simulink model "rov_ctrl_deploy"  (R2023b)
settings: Solver=FixedStepDiscrete  StartTime=0  StopTime=100  FixedStep=0.01  RelTol=1e-3
PreLoadFcn:
  | try, S=load('rovmodel75kg.mat'); catch, S=load('C:\Users\yhm\wb_hil\rovmodel75kg.mat'); end; fn=fieldnames(S); for k=1:numel(fn), assignin('base',fn{k},S.(fn{k})); end; M_nom=S.M; Ma_nom=S.Ma; DL_nom=S.DL; clear S fn k;
values from neighbouring files (symbols this model uses):
  I = [2.51  0  0; 0  3.38  0.01; 0  0.01  1.73]    [rovmodel75kg.mat]
  m = [75  0  0; 0  75  0; 0  0  75]    [rovmodel75kg.mat]
  Ma = [-20.392 0 0 0 0 0 0 -53.435 0 0 0 0 ... (36 elements, 6x6)]    [rovmodel75kg.mat]
  rg = [0 0 0]    [rovmodel75kg.mat]
undefined symbols (not defined in the file or in its folder): DiscIntNeverNeededParam
libraries: matrix_library x6, simulink x1
settings Model: Creator=yhm  LastModifiedBy=yhm
settings OptimizationCC: DefaultParameterBehavior=Inlined  EnhancedBackFolding=on  PassReuseOutputArgsAs=Individual arguments  ZeroExternalMemoryAtStartup=off  ZeroInternalMemoryAtStartup=off  OptimizeBlockOrder=speed  DifferentSizesBufferReuse=on  OptimizationCustomize=off  EfficientTunableParamExpr=on
settings DebuggingCC: ParameterTunabilityLossMsg=error
settings SFSimCC: MATLABDynamicMemAlloc=off
settings RTWCC: Description=Embedded Coder  SystemTargetFile=ert.tlc  TemplateMakefile=ert_default_tmf
settings CodeAppCC: ForceParamTrailComments=on  IgnoreCustomStorageClasses=off  OperatorAnnotations=on  SimulinkDataObjDesc=on  SFDataObjDesc=on  InsertBlockDesc=on
settings ERTTargetCC: TargetLangStandard=C99 (ISO)  GenerateSampleERTMain=on  InlinedParameterPlacement=NonHierarchical  ERTCustomFileTemplate=example_file_process.tlc

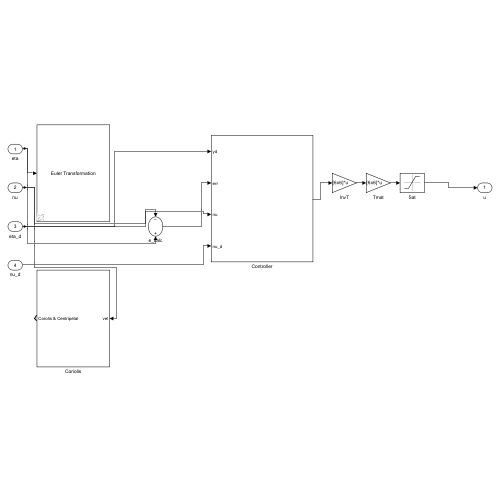
[thumbnail: Simulink's stored preview of the top-level diagram]
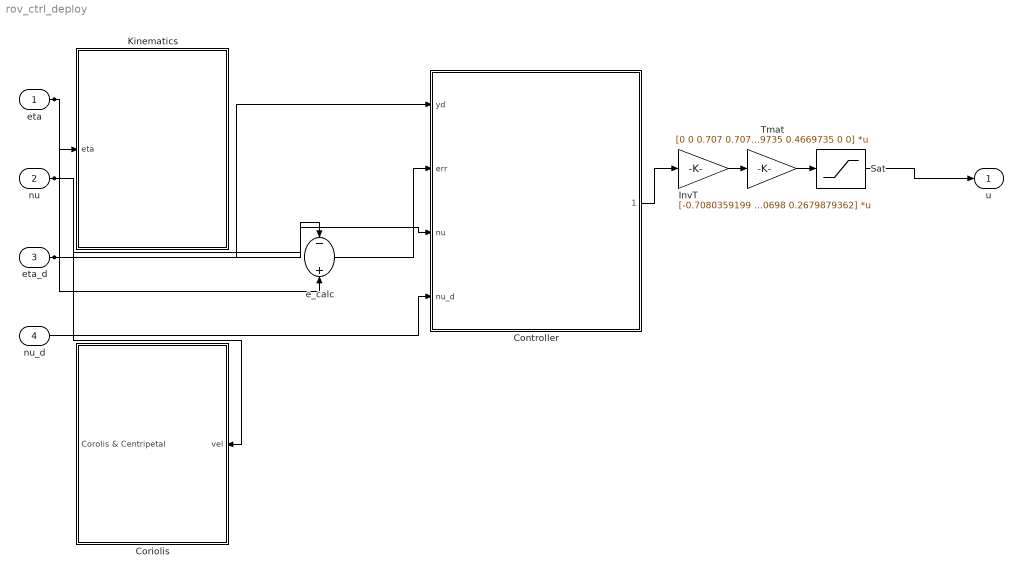
== system rov_ctrl_deploy ==
  eta : Inport  OutDataTypeStr=double  PortDimensions=6
  nu : Inport  Port=2  OutDataTypeStr=double  PortDimensions=6
  eta_d : Inport  Port=3  OutDataTypeStr=double  PortDimensions=6
  nu_d : Inport  Port=4  OutDataTypeStr=double  PortDimensions=6
  Controller : Subsystem
  Coriolis : Subsystem
  InvT : Gain  Gain=[-0.7080359199 -0.4427626243 0.05838623729 9.795787713e-17 1.644682741 -0.6703446242;-0.7080359199 0.4427626243 0.05838623729 3.755136333e-16 1.644682741 0.6703446242;0.7072135785 0.2644509542 1.700029006e-16 3.936371478e-16 -9.992007222e-16 -0.6703446242;0.7072135785 -0.2644509542 4.510281038e-17 1.299591795e-16 -1.054711873e-15 0.6703446242;0.5005813953 -0.1770060319 0.4587209302 -1.818181818 -1.162790698 -0.2679879362;0.5005813953 0.1770060319 0.4587209302 1.818181818 -1.162790698 0.2679879362]  Multiplication=Matrix(K*u)
  Kinematics : Subsystem  AncestorBlock=rov_design_analysis/Scope Utilities/Euler Transformation
      mask Display: disp('Euler Transformation')
  Sat : Saturate  UpperLimit=100  LowerLimit=-100
  Tmat : Gain  Gain=[0 0 0.707 0.707 0 0;-0.707 0.707 0.707 -0.707 0 0;0.707 0.707 0 0 1 1;0.1099385 -0.1099385 0 0 -0.275 0.275;0.2789115 0.2789115 0.3043635 0.3043635 -0.0355 -0.0355;-0.2789115 0.2789115 -0.4669735 0.4669735 0 0]  Multiplication=Matrix(K*u)
  e_calc : Sum  Inputs=-+
  u : Outport  PortDimensions=6
  wires:
  eta/1 -> Kinematics/1(eta), e_calc/2
  nu/1 -> Coriolis/1(vel), Controller/3(nu)
  eta_d/1 -> e_calc/1, Controller/1(yd)
  nu_d/1 -> Controller/4(nu_d)
  e_calc/1 -> Controller/2(err)
  Controller/1(" ") -> InvT/1
  InvT/1 -> Tmat/1
  Tmat/1 -> Sat/1
  Sat/1 -> u/1

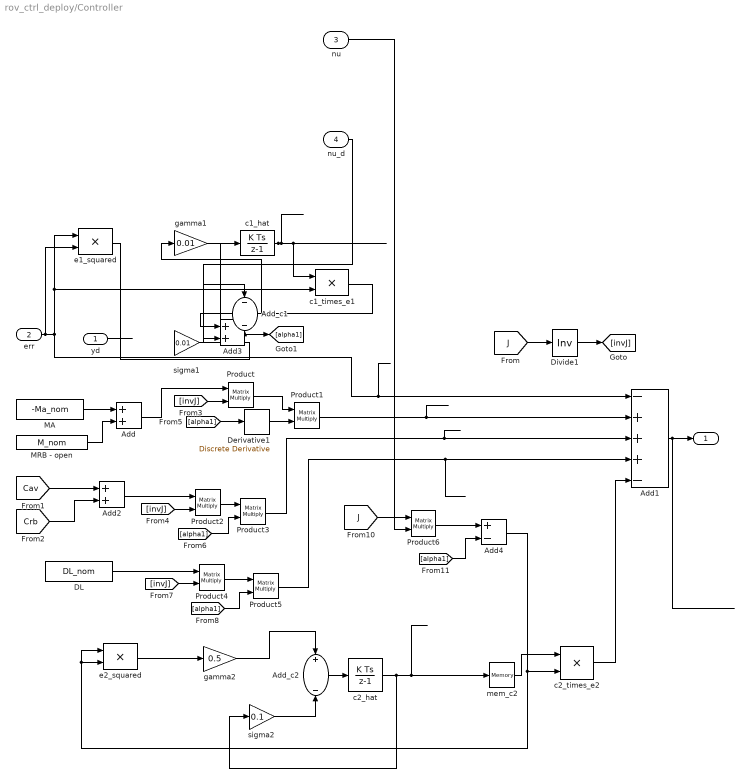
== system rov_ctrl_deploy/Controller ==
  yd : Inport  PortDimensions=6
  err : Inport  Port=2  PortDimensions=6
  nu : Inport  Port=3  OutDataTypeStr=double  PortDimensions=6
  nu_d : Inport  Port=4  OutDataTypeStr=double  PortDimensions=6
  Add : Sum
  Add1 : Sum  Inputs=-+++-
  Add2 : Sum
  Add3 : Sum
  Add4 : Sum  Inputs=+-
  Add_c1 : Sum  Inputs=--
  Add_c2 : Sum  Inputs=+-
  DL : Constant  Value=DL_nom
  Derivative1 : simulink/Discrete/Discrete Derivative  gainval=1  ICPrevScaledInput=0.0  OutMin=[]  OutMax=[]  OutDataType=fixdt(1, 16)  OutScaling=2^-10  DoSatur=off
      link override UD: SampleTime=0.01
  Divide1 : Product  Inputs=/  Multiplication=Matrix(*)
  MA : Constant  Value=-Ma_nom
  MRB - open : Constant  Value=M_nom
  Product{,1..6} (7 alike) : Product  Multiplication=Matrix(*)
  c1_hat : DiscreteIntegrator  InitialCondition=-3  SampleTime=0.01  ICPrevOutput=DiscIntNeverNeededParam  ICPrevScaledInput=DiscIntNeverNeededParam
  c1_times_e1 : Product
  c2_hat : DiscreteIntegrator  InitialCondition=5  SampleTime=0.01  ICPrevOutput=DiscIntNeverNeededParam  ICPrevScaledInput=DiscIntNeverNeededParam
  c2_times_e2 : Product
  e1_squared : Product
  e2_squared : Product
  gamma1 : Gain  Gain=0.01
  gamma2 : Gain  Gain=0.5
  mem_c2 : Memory  InitialCondition=5
  sigma1 : Gain  Gain=0.01
  sigma2 : Gain  Gain=0.1
  " " : Outport  PortDimensions=6
  wires:
  gamma1/1 -> c1_hat/1
  Add_c1/1 -> gamma1/1
  e1_squared/1 -> Add_c1/2
  sigma1/1 -> Add_c1/1
  c2_hat/1 -> sigma2/1, mem_c2/1
  e2_squared/1 -> gamma2/1
  mem_c2/1 -> c2_times_e2/1
  Add4/1 -> c2_times_e2/2, e2_squared/2, e2_squared/1
  c2_times_e2/1 -> Add1/5
  Add1/1 -> " "/1
  c1_times_e1/1 -> Add3/1
  Add_c2/1 -> c2_hat/1
  sigma2/1 -> Add_c2/2
  gamma2/1 -> Add_c2/1
  c1_hat/1 -> sigma1/1, c1_times_e1/1
  err/1 -> e1_squared/2, Add1/1, c1_times_e1/2, e1_squared/1
  Product1/1 -> Add1/2
  Product3/1 -> Add1/3
  Product5/1 -> Add1/4
  [alpha1] -> Add4/2
  Product6/1 -> Add4/1
  [J] -> Product6/1
  [alpha1] -> Product5/2
  Product4/1 -> Product5/1
  [invJ] -> Product4/2
  DL/1 -> Product4/1
  [alpha1] -> Derivative1/1
  Derivative1/1 -> Product1/2
  [alpha1] -> Product3/2
  Add3/1 -> [alpha1]
  Product2/1 -> Product3/1
  [invJ] -> Product2/2
  Add2/1 -> Product2/1
  [invJ] -> Product/2
  Divide1/1 -> [invJ]
  [Cav] -> Add2/1
  [Crb] -> Add2/2
  Product/1 -> Product1/1
  yd/1 -> ?
  Add/1 -> Product/1
  [J] -> Divide1/1
  MRB - open/1 -> Add/2
  MA/1 -> Add/1
  nu/1 -> Product6/2
  nu_d/1 -> Add3/2

== system rov_ctrl_deploy/Coriolis ==
  vel : Inport
  Add2 : Sum
  Centripetal & Coriolis : Subsystem  AncestorBlock=rov_design_analysis/ROV Models/1. Six DOF RRC ROV II/Centripetal & Coriolis
      mask Display: disp('CRB')
  Centripetal & Coriolis1 : Subsystem  AncestorBlock=rov_design_analysis/ROV Models/1. Six DOF RRC ROV II/Centripetal & Coriolis
      mask Display: disp('CA')
  Product5 : Product  Multiplication=Matrix(*)
  Subsystem : Subsystem
      mask Display: disp('CRB(v)')
  Corolis & Centripetal : Outport
  tag scope: Cav=global, Crb=global
  wires:
  Centripetal & Coriolis1/1(Ca) -> Add2/1, [Cav]
  Subsystem/1(Out1) -> [Crb], Add2/2
  Product5/1 -> Corolis & Centripetal/1
  vel/1 -> Centripetal & Coriolis1/1(vel), Subsystem/1(In1), Product5/2
  Add2/1 -> Product5/1

== system rov_ctrl_deploy/Kinematics ==
  eta : Inport
  Demux1 : Demux  Outputs=2
      settings: DisplayOption=none
  Matrix Concatenate6 : Concatenate  NumInputs=6  Mode=Multidimensional array
  Subsystem : Subsystem
      mask Display: disp('Transformation J first Row')
  Subsystem1 : Subsystem
      mask Display: disp('Transformation J second Row')
  Subsystem2 : Subsystem
      mask Display: disp('Transformation J third Row')
  Subsystem3 : Subsystem
      mask Display: disp('Transformation J fourth Row')
  Subsystem4 : Subsystem
      mask Display: disp('Transformation J fifth Row')
  Subsystem5 : Subsystem
      mask Display: disp('Transformation J sixth Row')
  tag scope: J=global
  wires:
  ? -> ?
  ? -> ?
  Subsystem5/1(Out1) -> Matrix Concatenate6/6
  Subsystem4/1(Out1) -> Matrix Concatenate6/5
  Subsystem3/1(Out1) -> Matrix Concatenate6/4
  Subsystem2/1(Out1) -> Matrix Concatenate6/3
  Subsystem1/1(Out1) -> Matrix Concatenate6/2
  Demux1/2 -> Subsystem5/1(In1), Subsystem4/1(In1), Subsystem3/1(In1), Subsystem2/1(In1), Subsystem1/1(In1), Subsystem/1(In1)
  Subsystem/1(Out1) -> Matrix Concatenate6/1
  Matrix Concatenate6/1 -> [J]
  ? -> ?
  Demux1/1 -> ?
  eta/1 -> Demux1/1

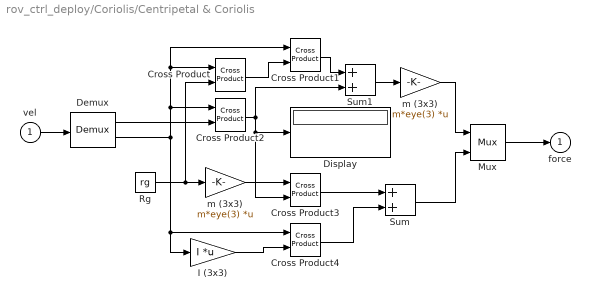
== system rov_ctrl_deploy/Coriolis/Centripetal & Coriolis ==
  vel : Inport
  Cross Product{,1..4} (5 alike) : matrix_library/Cross Product
  Demux : Demux  Outputs=2
      settings: DisplayOption=none
  Display : Display
  "I (3x3) " : Gain  Gain=I  Multiplication=Matrix(K*u)  SaturateOnIntegerOverflow=on  OutDataTypeStr=Inherit: Same as input  ParamDataTypeStr=Inherit: Same as input
  Mux : Mux  Inputs=2
  Rg : Constant  Value=rg
  Sum : Sum  InputSameDT=on  SaturateOnIntegerOverflow=on  OutDataTypeStr=Inherit: Same as first input
  Sum1 : Sum  InputSameDT=on  SaturateOnIntegerOverflow=on  OutDataTypeStr=Inherit: Same as first input
  m (3x3) : Gain  Gain=m*eye(3)  Multiplication=Matrix(K*u)  SaturateOnIntegerOverflow=on  OutDataTypeStr=Inherit: Same as input  ParamDataTypeStr=Inherit: Same as input
  "m (3x3) " : Gain  Gain=m*eye(3)  Multiplication=Matrix(K*u)  SaturateOnIntegerOverflow=on  OutDataTypeStr=Inherit: Same as input  ParamDataTypeStr=Inherit: Same as input
  force : Outport  InitialOutput=0
  wires:
  Demux/1 -> Cross Product2/2
  Cross Product2/1 -> Sum1/2, Display/1, Cross Product3/2
  "I (3x3) "/1 -> Cross Product4/2
  Rg/1 -> "m (3x3) "/1, Cross Product/2
  Demux/2 -> "I (3x3) "/1, Cross Product4/1, Cross Product/1, Cross Product1/1, Cross Product2/1
  Mux/1 -> force/1
  Sum/1 -> Mux/2
  m (3x3)/1 -> Mux/1
  vel/1 -> Demux/1
  Sum1/1 -> m (3x3)/1
  Cross Product1/1 -> Sum1/1
  Cross Product/1 -> Cross Product1/2
  Cross Product3/1 -> Sum/1
  "m (3x3) "/1 -> Cross Product3/1
  Cross Product4/1 -> Sum/2

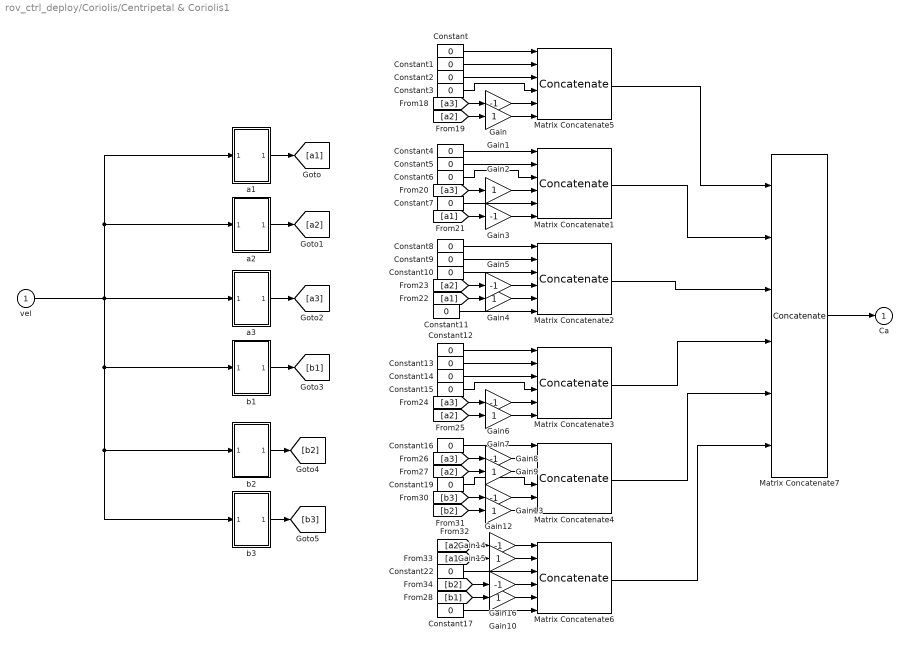
== system rov_ctrl_deploy/Coriolis/Centripetal & Coriolis1 ==
  vel : Inport
  Constant{,1..17,19,22} (20 alike) : Constant  Value=0
  Gain{,3,5..6,8,12,14,16} (8 alike) : Gain  Gain=-1
  Gain{1..2,4,7,9..10,13,15} (8 alike) : Gain
  Matrix Concatenate{1..6} (6 alike) : Concatenate  NumInputs=6  Mode=Multidimensional array  ConcatenateDimension=2
  Matrix Concatenate7 : Concatenate  NumInputs=6  Mode=Multidimensional array
  a1 : Subsystem
      mask Display: disp('Row 1')
  a2 : Subsystem
      mask Display: disp('Row 2')
  a3 : Subsystem
      mask Display: disp('Row 1')
  b1 : Subsystem
      mask Display: disp('Row 2')
  b2 : Subsystem
      mask Display: disp('Row 1')
  b3 : Subsystem
      mask Display: disp('Row 2')
  Ca : Outport  InitialOutput=0
  wires:
  Matrix Concatenate7/1 -> Ca/1
  Matrix Concatenate6/1 -> Matrix Concatenate7/6
  Matrix Concatenate4/1 -> Matrix Concatenate7/5
  Matrix Concatenate3/1 -> Matrix Concatenate7/4
  Matrix Concatenate2/1 -> Matrix Concatenate7/3
  Matrix Concatenate1/1 -> Matrix Concatenate7/2
  Matrix Concatenate5/1 -> Matrix Concatenate7/1
  Constant17/1 -> Matrix Concatenate6/6
  [b2] -> Gain16/1
  Gain16/1 -> Matrix Concatenate6/4
  [a1] -> Gain15/1
  Gain15/1 -> Matrix Concatenate6/2
  [a2] -> Gain14/1
  Gain14/1 -> Matrix Concatenate6/1
  [b2] -> Gain13/1
  Gain13/1 -> Matrix Concatenate4/6
  Gain12/1 -> Matrix Concatenate4/5
  [b3] -> Gain12/1
  Gain9/1 -> Matrix Concatenate4/3
  Constant11/1 -> Matrix Concatenate2/6
  Gain5/1 -> Matrix Concatenate2/4
  Constant7/1 -> Matrix Concatenate1/5
  Constant6/1 -> Matrix Concatenate1/3
  Gain2/1 -> Matrix Concatenate1/4
  Gain10/1 -> Matrix Concatenate6/5
  [b1] -> Gain10/1
  Constant22/1 -> Matrix Concatenate6/3
  Constant16/1 -> Matrix Concatenate4/1
  [a2] -> Gain9/1
  Constant19/1 -> Matrix Concatenate4/4
  [a3] -> Gain8/1
  Gain8/1 -> Matrix Concatenate4/2
  Constant12/1 -> Matrix Concatenate3/1
  Gain6/1 -> Matrix Concatenate3/5
  Gain7/1 -> Matrix Concatenate3/6
  [a2] -> Gain7/1
  Constant15/1 -> Matrix Concatenate3/4
  [a3] -> Gain6/1
  Constant13/1 -> Matrix Concatenate3/2
  Constant14/1 -> Matrix Concatenate3/3
  Constant8/1 -> Matrix Concatenate2/1
  Gain4/1 -> Matrix Concatenate2/5
  [a2] -> Gain5/1
  [a1] -> Gain4/1
  Constant9/1 -> Matrix Concatenate2/2
  Constant10/1 -> Matrix Concatenate2/3
  Constant4/1 -> Matrix Concatenate1/1
  Gain3/1 -> Matrix Concatenate1/6
  [a1] -> Gain3/1
  [a3] -> Gain2/1
  Constant5/1 -> Matrix Concatenate1/2
  [a2] -> Gain1/1
  [a3] -> Gain/1
  Constant3/1 -> Matrix Concatenate5/4
  Constant2/1 -> Matrix Concatenate5/3
  Constant1/1 -> Matrix Concatenate5/2
  Gain1/1 -> Matrix Concatenate5/6
  Gain/1 -> Matrix Concatenate5/5
  Constant/1 -> Matrix Concatenate5/1
  b3/1(Out1) -> [b3]
  b1/1(Out1) -> [b1]
  a2/1(Out1) -> [a2]
  a3/1(Out1) -> [a3]
  b2/1(Out1) -> [b2]
  a1/1(Out1) -> [a1]
  vel/1 -> a2/1(In1), a1/1(In1), a3/1(In1), b1/1(In1), b2/1(In1), b3/1(In1)

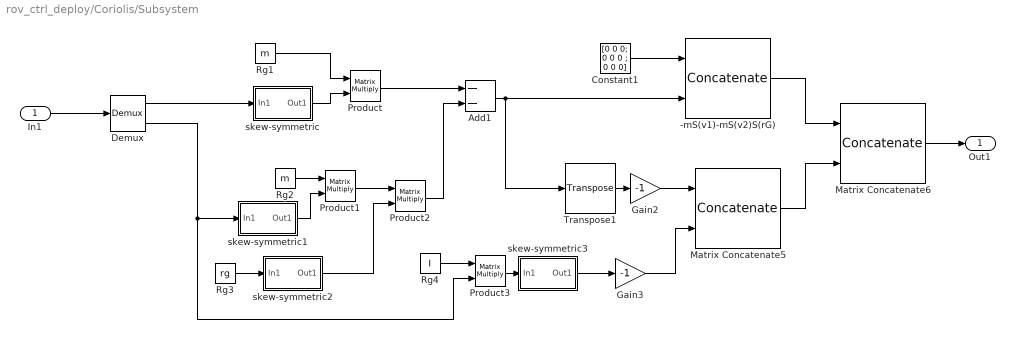
== system rov_ctrl_deploy/Coriolis/Subsystem ==
  In1 : Inport
  -mS(v1)-mS(v2)S(rG) : Concatenate  Mode=Multidimensional array  ConcatenateDimension=2
  Add1 : Sum  Inputs=--
  Constant1 : Constant  Value=[0 0 0; 0 0 0 ; 0 0 0]
  Demux : Demux  Outputs=2
      settings: DisplayOption=none
  Gain2 : Gain  Gain=-1
  Gain3 : Gain  Gain=-1
  Matrix Concatenate5 : Concatenate  Mode=Multidimensional array  ConcatenateDimension=2
  Matrix Concatenate6 : Concatenate  Mode=Multidimensional array
  Product{,1..3} (4 alike) : Product  Multiplication=Matrix(*)
  Rg1 : Constant  Value=m
  Rg2 : Constant  Value=m
  Rg3 : Constant  Value=rg
  Rg4 : Constant  Value=I
  Transpose1 : matrix_library/Transpose
  skew-symmetric : Subsystem
  skew-symmetric1 : Subsystem
  skew-symmetric2 : Subsystem
  skew-symmetric3 : Subsystem
  Out1 : Outport
  wires:
  Product1/1 -> Product2/1
  Product/1 -> Add1/1
  Rg1/1 -> Product/1
  -mS(v1)-mS(v2)S(rG)/1 -> Matrix Concatenate6/1
  Demux/1 -> skew-symmetric/1(In1)
  skew-symmetric/1(Out1) -> Product/2
  skew-symmetric2/1(Out1) -> Product2/2
  Transpose1/1 -> Gain2/1
  skew-symmetric3/1(Out1) -> Gain3/1
  Matrix Concatenate6/1 -> Out1/1
  Gain2/1 -> Matrix Concatenate5/1
  Product2/1 -> Add1/2
  Add1/1 -> Transpose1/1, -mS(v1)-mS(v2)S(rG)/2
  Gain3/1 -> Matrix Concatenate5/2
  Demux/2 -> skew-symmetric1/1(In1), Product3/2
  Constant1/1 -> -mS(v1)-mS(v2)S(rG)/1
  Rg4/1 -> Product3/1
  Matrix Concatenate5/1 -> Matrix Concatenate6/2
  Rg3/1 -> skew-symmetric2/1(In1)
  skew-symmetric1/1(Out1) -> Product1/2
  Product3/1 -> skew-symmetric3/1(In1)
  Rg2/1 -> Product1/1
  In1/1 -> Demux/1

== system rov_ctrl_deploy/Kinematics/Subsystem ==
  In1 : Inport
  -sZ.cX+cZ.sY.sX : Fcn  Expr=-sin(u[3])*cos(u[1]) + cos(u[3])*sin(u[2])*sin(u[1])
  Constant : Constant  Value=0
  Matrix Concatenate : Concatenate  NumInputs=6  Mode=Multidimensional array  ConcatenateDimension=2
  cY.cZ : Fcn  Expr=cos(u[3]) * cos(u[2])
  sZ.sX+cZ.cX.sY : Fcn  Expr=sin(u[3])*sin(u[1]) + cos(u[3])*cos(u[1])*sin(u[2])
  Out1 : Outport
  wires:
  In1/1 -> cY.cZ/1, -sZ.cX+cZ.sY.sX/1, sZ.sX+cZ.cX.sY/1
  -sZ.cX+cZ.sY.sX/1 -> Matrix Concatenate/2
  sZ.sX+cZ.cX.sY/1 -> Matrix Concatenate/3
  Matrix Concatenate/1 -> Out1/1
  cY.cZ/1 -> Matrix Concatenate/1
  Constant/1 -> Matrix Concatenate/4, Matrix Concatenate/5, Matrix Concatenate/6

== system rov_ctrl_deploy/Kinematics/Subsystem1 ==
  In1 : Inport
  -cZ.sX+sY.sZ.cX : Fcn  Expr=-cos(u[3])*sin(u[1]) + sin(u[2])*sin(u[3])*cos(u[1])
  Constant1 : Constant  Value=0
  Matrix Concatenate1 : Concatenate  NumInputs=6  Mode=Multidimensional array  ConcatenateDimension=2
  cY.sZ : Fcn  Expr=sin(u[3]) * cos(u[2])
  cZ.cX+sX.sY.sZ : Fcn  Expr=cos(u[3])*cos(u[1]) + sin(u[1])*sin(u[2])*sin(u[3])
  Out1 : Outport
  wires:
  In1/1 -> cY.sZ/1, cZ.cX+sX.sY.sZ/1, -cZ.sX+sY.sZ.cX/1
  Constant1/1 -> Matrix Concatenate1/4, Matrix Concatenate1/5, Matrix Concatenate1/6
  cZ.cX+sX.sY.sZ/1 -> Matrix Concatenate1/2
  -cZ.sX+sY.sZ.cX/1 -> Matrix Concatenate1/3
  Matrix Concatenate1/1 -> Out1/1
  cY.sZ/1 -> Matrix Concatenate1/1

== system rov_ctrl_deploy/Kinematics/Subsystem2 ==
  In1 : Inport
  -sY : Fcn  Expr=-sin(u[2])
  Constant2 : Constant  Value=0
  Matrix Concatenate2 : Concatenate  NumInputs=6  Mode=Multidimensional array  ConcatenateDimension=2
  cY.cX : Fcn  Expr=cos(u[2])*cos(u[1])
  cY.sX : Fcn  Expr=cos(u[2])*sin(u[1])
  Out1 : Outport
  wires:
  In1/1 -> -sY/1, cY.sX/1, cY.cX/1
  -sY/1 -> Matrix Concatenate2/1
  cY.cX/1 -> Matrix Concatenate2/3
  cY.sX/1 -> Matrix Concatenate2/2
  Constant2/1 -> Matrix Concatenate2/4, Matrix Concatenate2/5, Matrix Concatenate2/6
  Matrix Concatenate2/1 -> Out1/1

== system rov_ctrl_deploy/Kinematics/Subsystem3 ==
  In1 : Inport
  1 : Fcn  Expr=1
  Constant3 : Constant  Value=0
  Matrix Concatenate3 : Concatenate  NumInputs=6  Mode=Multidimensional array  ConcatenateDimension=2
  cX.tY : Fcn  Expr=cos(u[1])*tan(u[2])
  sX.tY : Fcn  Expr=sin(u[1])*tan(u[2])
  Out1 : Outport
  wires:
  In1/1 -> 1/1, sX.tY/1, cX.tY/1
  Matrix Concatenate3/1 -> Out1/1
  Constant3/1 -> Matrix Concatenate3/1, Matrix Concatenate3/2, Matrix Concatenate3/3
  1/1 -> Matrix Concatenate3/4
  sX.tY/1 -> Matrix Concatenate3/5
  cX.tY/1 -> Matrix Concatenate3/6

== system rov_ctrl_deploy/Kinematics/Subsystem4 ==
  In1 : Inport
  -sX : Fcn  Expr=-sin(u[1])
  0 : Fcn  Expr=0
  Constant4 : Constant  Value=0
  Dot Product1 : Subsystem
  Matrix Concatenate4 : Concatenate  NumInputs=6  Mode=Multidimensional array  ConcatenateDimension=2
  cX : Fcn  Expr=cos(u[1])
  Out1 : Outport
  wires:
  -sX/1 -> Matrix Concatenate4/6
  Constant4/1 -> Matrix Concatenate4/1, Matrix Concatenate4/2, Matrix Concatenate4/3
  Matrix Concatenate4/1 -> Out1/1
  0/1 -> Matrix Concatenate4/4
  cX/1 -> Matrix Concatenate4/5
  In1/1 -> 0/1, cX/1, -sX/1

== system rov_ctrl_deploy/Kinematics/Subsystem5 ==
  In1 : Inport
  2 : Fcn  Expr=0
  Constant5 : Constant  Value=0
  Matrix Concatenate5 : Concatenate  NumInputs=6  Mode=Multidimensional array  ConcatenateDimension=2
  cX/cY : Fcn  Expr=cos(u[1])/cos(u[2])
  sX/cY : Fcn  Expr=sin(u[1])/cos(u[2])
  Out1 : Outport
  wires:
  Matrix Concatenate5/1 -> Out1/1
  sX/cY/1 -> Matrix Concatenate5/5
  2/1 -> Matrix Concatenate5/4
  In1/1 -> 2/1, sX/cY/1, cX/cY/1
  cX/cY/1 -> Matrix Concatenate5/6
  Constant5/1 -> Matrix Concatenate5/1, Matrix Concatenate5/2, Matrix Concatenate5/3

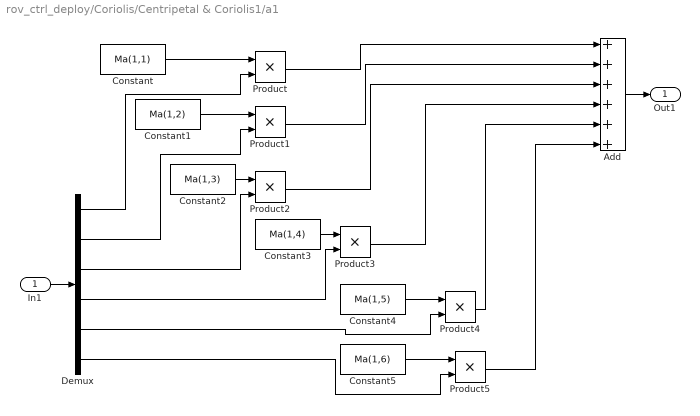
== system rov_ctrl_deploy/Coriolis/Centripetal & Coriolis1/a1 ==
  In1 : Inport
  Add : Sum  Inputs=++++++
  Constant : Constant  Value=Ma(1,1)
  Constant1 : Constant  Value=Ma(1,2)
  Constant2 : Constant  Value=Ma(1,3)
  Constant3 : Constant  Value=Ma(1,4)
  Constant4 : Constant  Value=Ma(1,5)
  Constant5 : Constant  Value=Ma(1,6)
  Demux : Demux  Outputs=6
  Product{,1..5} (6 alike) : Product  RndMeth=Zero
  Out1 : Outport
  wires:
  In1/1 -> Demux/1
  Add/1 -> Out1/1
  Constant/1 -> Product/1
  Product/1 -> Add/1
  Constant1/1 -> Product1/1
  Product1/1 -> Add/2
  Constant2/1 -> Product2/1
  Product2/1 -> Add/3
  Constant3/1 -> Product3/1
  Product3/1 -> Add/4
  Constant4/1 -> Product4/1
  Product4/1 -> Add/5
  Constant5/1 -> Product5/1
  Product5/1 -> Add/6
  Demux/6 -> Product5/2
  Demux/5 -> Product4/2
  Demux/4 -> Product3/2
  Demux/3 -> Product2/2
  Demux/2 -> Product1/2
  Demux/1 -> Product/2

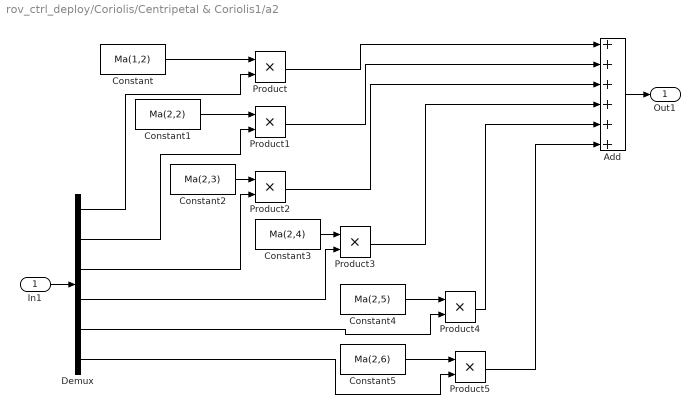
== system rov_ctrl_deploy/Coriolis/Centripetal & Coriolis1/a2 ==
  In1 : Inport
  Add : Sum  Inputs=++++++
  Constant : Constant  Value=Ma(1,2)
  Constant1 : Constant  Value=Ma(2,2)
  Constant2 : Constant  Value=Ma(2,3)
  Constant3 : Constant  Value=Ma(2,4)
  Constant4 : Constant  Value=Ma(2,5)
  Constant5 : Constant  Value=Ma(2,6)
  Demux : Demux  Outputs=6
  Product{,1..5} (6 alike) : Product  RndMeth=Zero
  Out1 : Outport
  wires:
  In1/1 -> Demux/1
  Add/1 -> Out1/1
  Constant/1 -> Product/1
  Product/1 -> Add/1
  Constant1/1 -> Product1/1
  Product1/1 -> Add/2
  Constant2/1 -> Product2/1
  Product2/1 -> Add/3
  Constant3/1 -> Product3/1
  Product3/1 -> Add/4
  Constant4/1 -> Product4/1
  Product4/1 -> Add/5
  Constant5/1 -> Product5/1
  Product5/1 -> Add/6
  Demux/6 -> Product5/2
  Demux/5 -> Product4/2
  Demux/4 -> Product3/2
  Demux/3 -> Product2/2
  Demux/2 -> Product1/2
  Demux/1 -> Product/2

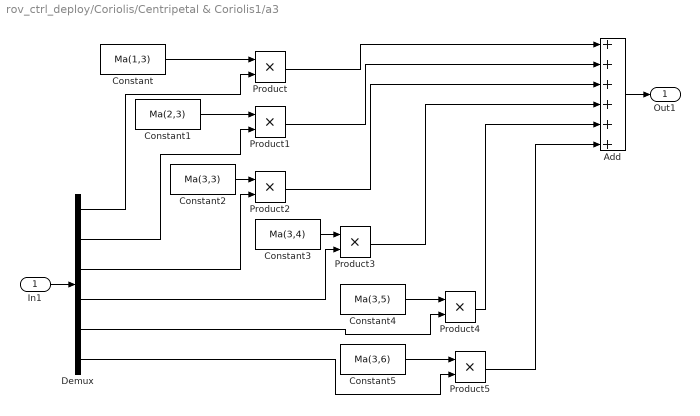
== system rov_ctrl_deploy/Coriolis/Centripetal & Coriolis1/a3 ==
  In1 : Inport
  Add : Sum  Inputs=++++++
  Constant : Constant  Value=Ma(1,3)
  Constant1 : Constant  Value=Ma(2,3)
  Constant2 : Constant  Value=Ma(3,3)
  Constant3 : Constant  Value=Ma(3,4)
  Constant4 : Constant  Value=Ma(3,5)
  Constant5 : Constant  Value=Ma(3,6)
  Demux : Demux  Outputs=6
  Product{,1..5} (6 alike) : Product  RndMeth=Zero
  Out1 : Outport
  wires:
  In1/1 -> Demux/1
  Add/1 -> Out1/1
  Constant/1 -> Product/1
  Product/1 -> Add/1
  Constant1/1 -> Product1/1
  Product1/1 -> Add/2
  Constant2/1 -> Product2/1
  Product2/1 -> Add/3
  Constant3/1 -> Product3/1
  Product3/1 -> Add/4
  Constant4/1 -> Product4/1
  Product4/1 -> Add/5
  Constant5/1 -> Product5/1
  Product5/1 -> Add/6
  Demux/6 -> Product5/2
  Demux/5 -> Product4/2
  Demux/4 -> Product3/2
  Demux/3 -> Product2/2
  Demux/2 -> Product1/2
  Demux/1 -> Product/2

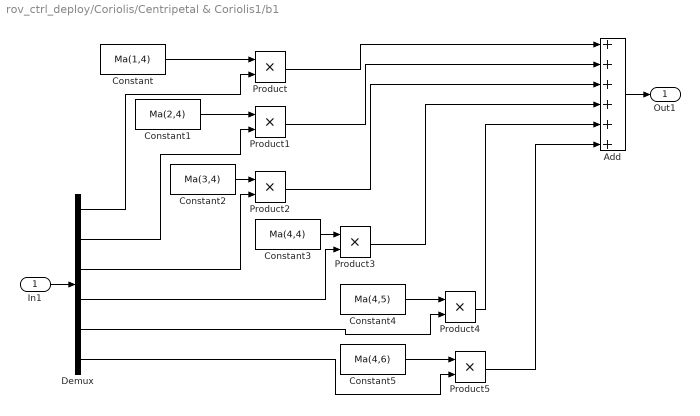
== system rov_ctrl_deploy/Coriolis/Centripetal & Coriolis1/b1 ==
  In1 : Inport
  Add : Sum  Inputs=++++++
  Constant : Constant  Value=Ma(1,4)
  Constant1 : Constant  Value=Ma(2,4)
  Constant2 : Constant  Value=Ma(3,4)
  Constant3 : Constant  Value=Ma(4,4)
  Constant4 : Constant  Value=Ma(4,5)
  Constant5 : Constant  Value=Ma(4,6)
  Demux : Demux  Outputs=6
  Product{,1..5} (6 alike) : Product  RndMeth=Zero
  Out1 : Outport
  wires:
  In1/1 -> Demux/1
  Add/1 -> Out1/1
  Constant/1 -> Product/1
  Product/1 -> Add/1
  Constant1/1 -> Product1/1
  Product1/1 -> Add/2
  Constant2/1 -> Product2/1
  Product2/1 -> Add/3
  Constant3/1 -> Product3/1
  Product3/1 -> Add/4
  Constant4/1 -> Product4/1
  Product4/1 -> Add/5
  Constant5/1 -> Product5/1
  Product5/1 -> Add/6
  Demux/6 -> Product5/2
  Demux/5 -> Product4/2
  Demux/4 -> Product3/2
  Demux/3 -> Product2/2
  Demux/2 -> Product1/2
  Demux/1 -> Product/2

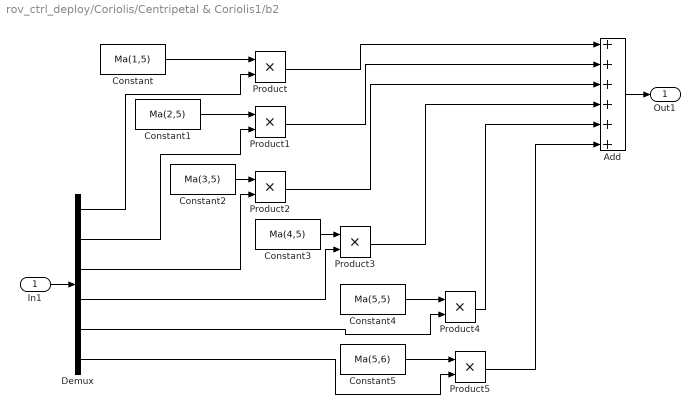
== system rov_ctrl_deploy/Coriolis/Centripetal & Coriolis1/b2 ==
  In1 : Inport
  Add : Sum  Inputs=++++++
  Constant : Constant  Value=Ma(1,5)
  Constant1 : Constant  Value=Ma(2,5)
  Constant2 : Constant  Value=Ma(3,5)
  Constant3 : Constant  Value=Ma(4,5)
  Constant4 : Constant  Value=Ma(5,5)
  Constant5 : Constant  Value=Ma(5,6)
  Demux : Demux  Outputs=6
  Product{,1..5} (6 alike) : Product  RndMeth=Zero
  Out1 : Outport
  wires:
  In1/1 -> Demux/1
  Add/1 -> Out1/1
  Constant/1 -> Product/1
  Product/1 -> Add/1
  Constant1/1 -> Product1/1
  Product1/1 -> Add/2
  Constant2/1 -> Product2/1
  Product2/1 -> Add/3
  Constant3/1 -> Product3/1
  Product3/1 -> Add/4
  Constant4/1 -> Product4/1
  Product4/1 -> Add/5
  Constant5/1 -> Product5/1
  Product5/1 -> Add/6
  Demux/6 -> Product5/2
  Demux/5 -> Product4/2
  Demux/4 -> Product3/2
  Demux/3 -> Product2/2
  Demux/2 -> Product1/2
  Demux/1 -> Product/2

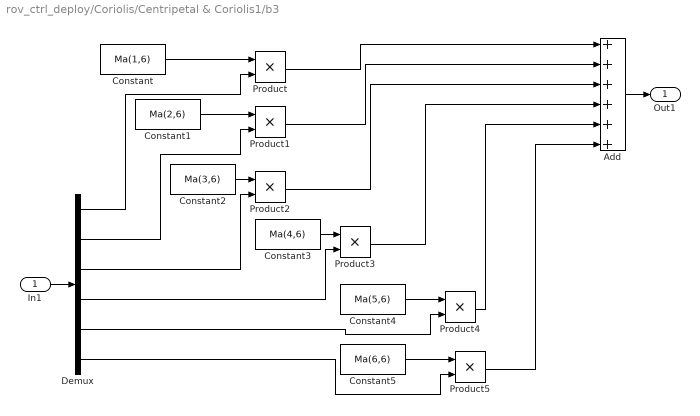
== system rov_ctrl_deploy/Coriolis/Centripetal & Coriolis1/b3 ==
  In1 : Inport
  Add : Sum  Inputs=++++++
  Constant : Constant  Value=Ma(1,6)
  Constant1 : Constant  Value=Ma(2,6)
  Constant2 : Constant  Value=Ma(3,6)
  Constant3 : Constant  Value=Ma(4,6)
  Constant4 : Constant  Value=Ma(5,6)
  Constant5 : Constant  Value=Ma(6,6)
  Demux : Demux  Outputs=6
  Product{,1..5} (6 alike) : Product  RndMeth=Zero
  Out1 : Outport
  wires:
  In1/1 -> Demux/1
  Add/1 -> Out1/1
  Constant/1 -> Product/1
  Product/1 -> Add/1
  Constant1/1 -> Product1/1
  Product1/1 -> Add/2
  Constant2/1 -> Product2/1
  Product2/1 -> Add/3
  Constant3/1 -> Product3/1
  Product3/1 -> Add/4
  Constant4/1 -> Product4/1
  Product4/1 -> Add/5
  Constant5/1 -> Product5/1
  Product5/1 -> Add/6
  Demux/6 -> Product5/2
  Demux/5 -> Product4/2
  Demux/4 -> Product3/2
  Demux/3 -> Product2/2
  Demux/2 -> Product1/2
  Demux/1 -> Product/2

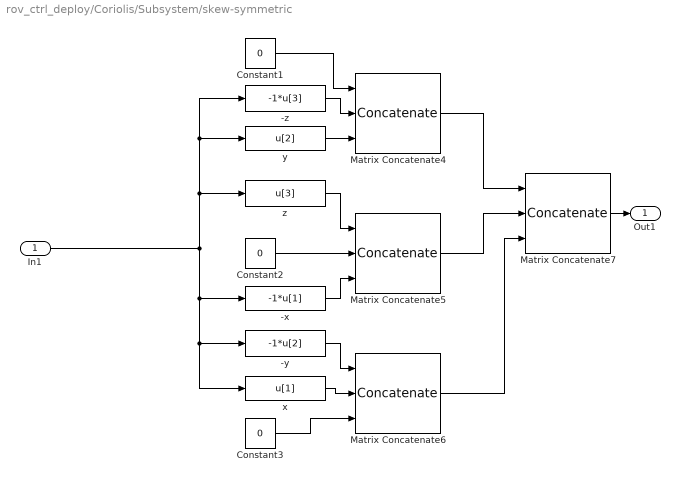
== system rov_ctrl_deploy/Coriolis/Subsystem/skew-symmetric ==
  In1 : Inport
  -x : Fcn  Expr=-1*u[1]
  -y : Fcn  Expr=-1*u[2]
  -z : Fcn  Expr=-1*u[3]
  Constant1 : Constant  Value=0
  Constant2 : Constant  Value=0
  Constant3 : Constant  Value=0
  Matrix Concatenate4 : Concatenate  NumInputs=3  Mode=Multidimensional array  ConcatenateDimension=2
  Matrix Concatenate5 : Concatenate  NumInputs=3  Mode=Multidimensional array  ConcatenateDimension=2
  Matrix Concatenate6 : Concatenate  NumInputs=3  Mode=Multidimensional array  ConcatenateDimension=2
  Matrix Concatenate7 : Concatenate  NumInputs=3  Mode=Multidimensional array
  x : Fcn  Expr=u[1]
  y : Fcn  Expr=u[2]
  z : Fcn  Expr=u[3]
  Out1 : Outport
  wires:
  Matrix Concatenate7/1 -> Out1/1
  In1/1 -> -x/1, -y/1, x/1, z/1, y/1, -z/1
  Matrix Concatenate5/1 -> Matrix Concatenate7/2
  Constant2/1 -> Matrix Concatenate5/2
  Constant3/1 -> Matrix Concatenate6/3
  y/1 -> Matrix Concatenate4/3
  -z/1 -> Matrix Concatenate4/2
  Constant1/1 -> Matrix Concatenate4/1
  x/1 -> Matrix Concatenate6/2
  Matrix Concatenate4/1 -> Matrix Concatenate7/1
  Matrix Concatenate6/1 -> Matrix Concatenate7/3
  -x/1 -> Matrix Concatenate5/3
  -y/1 -> Matrix Concatenate6/1
  z/1 -> Matrix Concatenate5/1

== system rov_ctrl_deploy/Coriolis/Subsystem/skew-symmetric1 ==
  In1 : Inport
  -x : Fcn  Expr=-1*u[1]
  -y : Fcn  Expr=-1*u[2]
  -z : Fcn  Expr=-1*u[3]
  Constant1 : Constant  Value=0
  Constant2 : Constant  Value=0
  Constant3 : Constant  Value=0
  Matrix Concatenate4 : Concatenate  NumInputs=3  Mode=Multidimensional array  ConcatenateDimension=2
  Matrix Concatenate5 : Concatenate  NumInputs=3  Mode=Multidimensional array  ConcatenateDimension=2
  Matrix Concatenate6 : Concatenate  NumInputs=3  Mode=Multidimensional array  ConcatenateDimension=2
  Matrix Concatenate7 : Concatenate  NumInputs=3  Mode=Multidimensional array
  x : Fcn  Expr=u[1]
  y : Fcn  Expr=u[2]
  z : Fcn  Expr=u[3]
  Out1 : Outport
  wires:
  Matrix Concatenate7/1 -> Out1/1
  In1/1 -> -x/1, -y/1, x/1, z/1, y/1, -z/1
  Matrix Concatenate5/1 -> Matrix Concatenate7/2
  Constant2/1 -> Matrix Concatenate5/2
  Constant3/1 -> Matrix Concatenate6/3
  y/1 -> Matrix Concatenate4/3
  -z/1 -> Matrix Concatenate4/2
  Constant1/1 -> Matrix Concatenate4/1
  x/1 -> Matrix Concatenate6/2
  Matrix Concatenate4/1 -> Matrix Concatenate7/1
  Matrix Concatenate6/1 -> Matrix Concatenate7/3
  -x/1 -> Matrix Concatenate5/3
  -y/1 -> Matrix Concatenate6/1
  z/1 -> Matrix Concatenate5/1

== system rov_ctrl_deploy/Coriolis/Subsystem/skew-symmetric2 ==
  In1 : Inport
  -x : Fcn  Expr=-1*u[1]
  -y : Fcn  Expr=-1*u[2]
  -z : Fcn  Expr=-1*u[3]
  Constant1 : Constant  Value=0
  Constant2 : Constant  Value=0
  Constant3 : Constant  Value=0
  Matrix Concatenate4 : Concatenate  NumInputs=3  Mode=Multidimensional array  ConcatenateDimension=2
  Matrix Concatenate5 : Concatenate  NumInputs=3  Mode=Multidimensional array  ConcatenateDimension=2
  Matrix Concatenate6 : Concatenate  NumInputs=3  Mode=Multidimensional array  ConcatenateDimension=2
  Matrix Concatenate7 : Concatenate  NumInputs=3  Mode=Multidimensional array
  x : Fcn  Expr=u[1]
  y : Fcn  Expr=u[2]
  z : Fcn  Expr=u[3]
  Out1 : Outport
  wires:
  Matrix Concatenate7/1 -> Out1/1
  In1/1 -> -x/1, -y/1, x/1, z/1, y/1, -z/1
  Matrix Concatenate5/1 -> Matrix Concatenate7/2
  Constant2/1 -> Matrix Concatenate5/2
  Constant3/1 -> Matrix Concatenate6/3
  y/1 -> Matrix Concatenate4/3
  -z/1 -> Matrix Concatenate4/2
  Constant1/1 -> Matrix Concatenate4/1
  x/1 -> Matrix Concatenate6/2
  Matrix Concatenate4/1 -> Matrix Concatenate7/1
  Matrix Concatenate6/1 -> Matrix Concatenate7/3
  -x/1 -> Matrix Concatenate5/3
  -y/1 -> Matrix Concatenate6/1
  z/1 -> Matrix Concatenate5/1

== system rov_ctrl_deploy/Coriolis/Subsystem/skew-symmetric3 ==
  In1 : Inport
  -x : Fcn  Expr=-1*u[1]
  -y : Fcn  Expr=-1*u[2]
  -z : Fcn  Expr=-1*u[3]
  Constant1 : Constant  Value=0
  Constant2 : Constant  Value=0
  Constant3 : Constant  Value=0
  Matrix Concatenate4 : Concatenate  NumInputs=3  Mode=Multidimensional array  ConcatenateDimension=2
  Matrix Concatenate5 : Concatenate  NumInputs=3  Mode=Multidimensional array  ConcatenateDimension=2
  Matrix Concatenate6 : Concatenate  NumInputs=3  Mode=Multidimensional array  ConcatenateDimension=2
  Matrix Concatenate7 : Concatenate  NumInputs=3  Mode=Multidimensional array
  x : Fcn  Expr=u[1]
  y : Fcn  Expr=u[2]
  z : Fcn  Expr=u[3]
  Out1 : Outport
  wires:
  Matrix Concatenate7/1 -> Out1/1
  In1/1 -> -x/1, -y/1, x/1, z/1, y/1, -z/1
  Matrix Concatenate5/1 -> Matrix Concatenate7/2
  Constant2/1 -> Matrix Concatenate5/2
  Constant3/1 -> Matrix Concatenate6/3
  y/1 -> Matrix Concatenate4/3
  -z/1 -> Matrix Concatenate4/2
  Constant1/1 -> Matrix Concatenate4/1
  x/1 -> Matrix Concatenate6/2
  Matrix Concatenate4/1 -> Matrix Concatenate7/1
  Matrix Concatenate6/1 -> Matrix Concatenate7/3
  -x/1 -> Matrix Concatenate5/3
  -y/1 -> Matrix Concatenate6/1
  z/1 -> Matrix Concatenate5/1

== system rov_ctrl_deploy/Kinematics/Subsystem4/Dot Product1 ==
